simulink model "FAST_11TO14mpers_testIPC"  (R2019b)
settings: Solver=FixedStepAuto  StartTime=0.0  StopTime=400  FixedStep=DT  RelTol=1e-3
values from neighbouring files (symbols this model uses):
  Drivetrain = struct    [dataDLR.m]
  OutList = OutTable.Properties.VariableNames    [initLPVParam.m]    (also in testCtrl.m; testOutList.m = cell(40, 1); testqLPV.m = cell(40, 1))
undefined symbols (not defined in the file or in its folder): RPM_Init, strmatch
settings Model: ExtModeTrigMode=oneshot  ExtModeArmWhenConnect=off  Creator=Hazim Namik  LastModifiedBy=ditt_aj
settings DataIOCC: LimitDataPoints=on  SaveFormat=Array  ReturnWorkspaceOutputs=off
settings OptimizationCC: BlockReduction=off  BooleanDataType=off  LifeSpan=inf
settings DebuggingCC: SaveWithParameterizedLinksMsg=none  UnderspecifiedInitializationDetection=Classic  MergeDetectMultiDrivingBlocksExec=none  SignalResolutionControl=TryResolveAllWithWarning  SFUnexpectedBacktrackingDiag=warning  SFNoUnconditionalDefaultTransitionDiag=warning  SFExecutionAtInitializationDiag=none  ArithmeticOperatorsInVariantConditions=warning
settings HardwareCC: ProdBitPerPointer=32  ProdBitPerSizeT=32  ProdBitPerPtrDiffT=32  ProdLargestAtomicFloat=None  ProdIntDivRoundTo=Undefined  ProdEndianess=Unspecified  ProdWordSize=32  ProdHWDeviceType=32-bit Generic  TargetUnknown=on
settings ModelReferenceCC: PropagateSignalLabelsOutOfModel=off
settings SFSimCC: SimUseLocalCustomCode=off  CustomCodeUndefinedFunction=UseInterfaceOnly
settings RTWCC: RTWUseLocalCustomCode=off
settings CodeAppCC: StateflowObjectComments=on
settings GRTTargetCC: TargetLangStandard=C89/C90 (ANSI)  GeneratePreprocessorConditionals=Disable all
settings ConfigComp: CovMetricSettings=dw  CovHtmlReporting=on  CovSaveCumulativeToWorkspaceVar=on  CovSaveSingleToWorkspaceVar=on  CovExternalEMLEnable=off

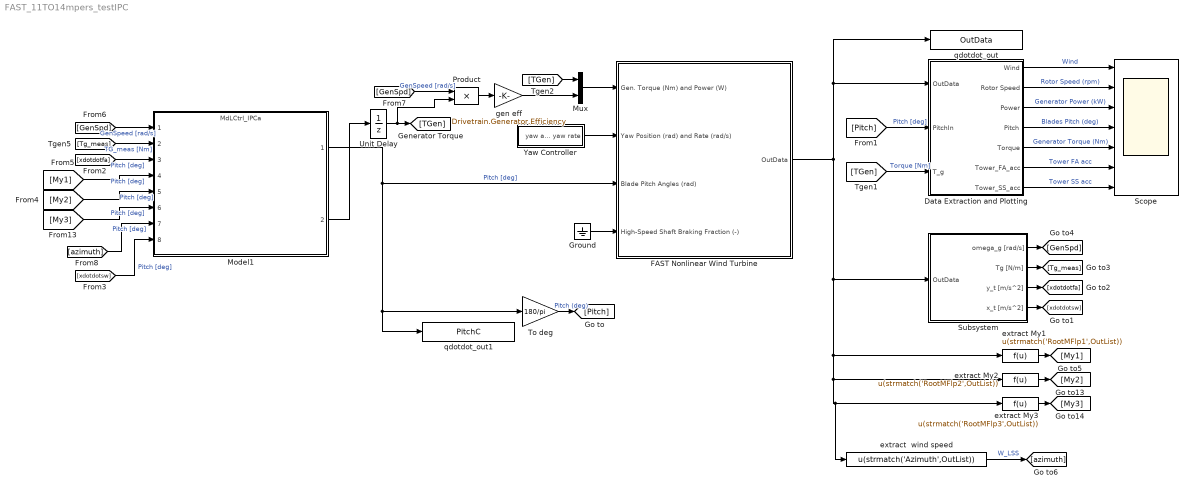
== system FAST_11TO14mpers_testIPC ==
  Data Extraction and Plotting : Subsystem
  FAST Nonlinear Wind Turbine : Subsystem  mask(FAST Nonlinear Wind Turbine){}
      mask help: This block contains the FAST S-Function.
      mask init:
      | clear FAST_SFunc
  Ground : Ground
  Model1 : ModelReference  ModelNameDialog=MdLCtrl_IPCa.slx  SimulationMode=Normal  ModelReferenceVersion=1.28
  Mux : Mux  Inputs=2
  Product : Product  RndMeth=Zero
  Scope : Scope  NumInputPorts=7
      settings: Tag=Scope
  Subsystem : Subsystem
  To deg : Gain  Gain=180/pi
  Unit Delay : UnitDelay  InitialCondition=RPM_Init*Drivetrain.Gearbox.Ratio  SampleTime=-1  HasFrameUpgradeWarning=on
  Yaw Controller : Subsystem
  extract  wind speed : Fcn  Expr=u(strmatch('Azimuth',OutList))
  extract My1 : Fcn  Expr=u(strmatch('RootMFlp1',OutList))
  extract My2 : Fcn  Expr=u(strmatch('RootMFlp2',OutList))
  extract My3 : Fcn  Expr=u(strmatch('RootMFlp3',OutList))
  gen eff : Gain  Gain=Drivetrain.Generator.Efficiency
  qdotdot_out : ToWorkspace  VariableName=OutData  SampleTime=-1
  qdotdot_out1 : ToWorkspace  VariableName=PitchC  SampleTime=-1
  wires:
  Mux/1 -> FAST Nonlinear Wind Turbine/1(Gen. Torque (Nm) and Power (W))
  Yaw Controller/1(yaw and yaw rate) -> FAST Nonlinear Wind Turbine/2(Yaw Position (rad) and Rate (rad/s))
  To deg/1 -> [Pitch]  "Pitch (deg)"
  gen eff/1 -> Mux/2
  Product/1 -> gen eff/1
  Data Extraction and Plotting/3(Power) -> Scope/3  "Generator Power (kW)"
  [Pitch] -> Data Extraction and Plotting/2(PitchIn)  "Pitch [deg]"
  Data Extraction and Plotting/1(Wind) -> Scope/1  "Wind"
  Data Extraction and Plotting/2(Rotor Speed) -> Scope/2  "Rotor Speed (rpm)"
  [TGen] -> Data Extraction and Plotting/3(T_g)  "Torque [Nm]"
  Data Extraction and Plotting/4(Pitch) -> Scope/4  "Blades Pitch (deg)"
  Data Extraction and Plotting/5(Torque) -> Scope/5  "Generator Torque (Nm)"
  Model1/2 -> Unit Delay/1
  Data Extraction and Plotting/6(Tower_FA_acc) -> Scope/6  "Tower FA acc"
  Data Extraction and Plotting/7(Tower_SS_acc) -> Scope/7  "Tower SS acc"
  Ground/1 -> FAST Nonlinear Wind Turbine/4(High-Speed Shaft Braking Fraction (-))
  [TGen] -> Mux/1
  Subsystem/1(omega_g [rad/s]) -> [GenSpd]
  Subsystem/3(y_t [m/s^2]) -> [xdotdotfa]
  Subsystem/4(x_t [m/s^2]) -> [xdotdotsw]
  [GenSpd] -> Model1/1  "GenSpeed [rad/s]"
  [Tg_meas] -> Model1/2  "TG_meas [Nm]"
  [xdotdotsw] -> Model1/8  "Pitch [deg]"
  [xdotdotfa] -> Model1/3  "Pitch [deg]"
  Subsystem/2(Tg [N/m]) -> [Tg_meas]
  [GenSpd] -> Product/1  "GenSpeed [rad/s]"
  Unit Delay/1 -> Product/2, [TGen]
  Model1/1 -> qdotdot_out1/1, To deg/1, FAST Nonlinear Wind Turbine/3(Blade Pitch Angles (rad))  "Pitch [deg]"
  FAST Nonlinear Wind Turbine/1(OutData) -> qdotdot_out/1, Data Extraction and Plotting/1(OutData), Subsystem/1(OutData), extract My1/1, extract My2/1, extract  wind speed/1, extract My3/1
  extract My2/1 -> [My2]
  extract My1/1 -> [My1]
  extract My3/1 -> [My3]
  [My1] -> Model1/4  "Pitch [deg]"
  [My2] -> Model1/5  "Pitch [deg]"
  [My3] -> Model1/6  "Pitch [deg]"
  extract  wind speed/1 -> [azimuth]  "W_LSS"
  [azimuth] -> Model1/7  "Pitch [deg]"

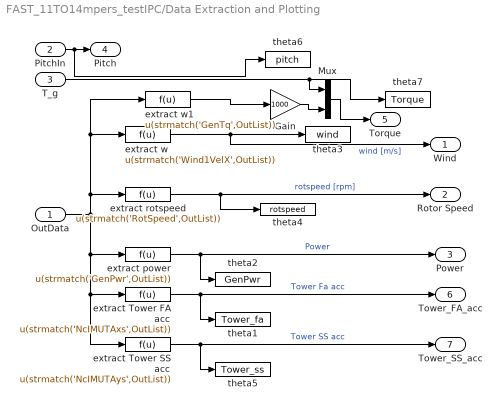
== system FAST_11TO14mpers_testIPC/Data Extraction and Plotting ==
  OutData : Inport
  PitchIn : Inport  Port=2
  T_g : Inport  Port=3
  Gain : Gain  Gain=1000
  Mux : Mux  Inputs=2
  extract Tower FA acc : Fcn  Expr=u(strmatch('NcIMUTAxs',OutList))
  extract Tower SS acc : Fcn  Expr=u(strmatch('NcIMUTAys',OutList))
  extract power : Fcn  Expr=u(strmatch('GenPwr',OutList))
  extract rotspeed : Fcn  Expr=u(strmatch('RotSpeed',OutList))
  extract w : Fcn  Expr=u(strmatch('Wind1VelX',OutList))
  extract w1 : Fcn  Expr=u(strmatch('GenTq',OutList))
  theta1 : ToWorkspace  VariableName=Tower_fa  SampleTime=-1
      settings: MaxDataPoints=Inf  Decimation=3
  theta2 : ToWorkspace  VariableName=GenPwr  SampleTime=-1
      settings: MaxDataPoints=Inf  Decimation=3
  theta3 : ToWorkspace  VariableName=wind  SampleTime=-1
      settings: MaxDataPoints=Inf  Decimation=3
  theta4 : ToWorkspace  VariableName=rotspeed  SampleTime=-1
      settings: MaxDataPoints=Inf  Decimation=3
  theta5 : ToWorkspace  VariableName=Tower_ss  SampleTime=-1
      settings: MaxDataPoints=Inf  Decimation=3
  theta6 : ToWorkspace  VariableName=pitch  SampleTime=-1
      settings: MaxDataPoints=Inf  Decimation=3
  theta7 : ToWorkspace  VariableName=Torque  SampleTime=-1
      settings: MaxDataPoints=Inf  Decimation=3
  Wind : Outport  VectorParamsAs1DForOutWhenUnconnected=off
  Rotor Speed : Outport  Port=2  VectorParamsAs1DForOutWhenUnconnected=off
  Power : Outport  Port=3  VectorParamsAs1DForOutWhenUnconnected=off
  Pitch : Outport  Port=4  VectorParamsAs1DForOutWhenUnconnected=off
  Torque : Outport  Port=5  VectorParamsAs1DForOutWhenUnconnected=off
  Tower_FA_acc : Outport  Port=6  VectorParamsAs1DForOutWhenUnconnected=off
  Tower_SS_acc : Outport  Port=7  VectorParamsAs1DForOutWhenUnconnected=off
  wires:
  extract w/1 -> Wind/1, theta3/1  "wind [m/s]"
  extract rotspeed/1 -> theta4/1, Rotor Speed/1  "rotspeed [rpm]"
  extract power/1 -> theta2/1, Power/1  "Power"
  PitchIn/1 -> theta6/1, Pitch/1
  T_g/1 -> Mux/1, theta7/1
  extract Tower FA acc/1 -> theta1/1, Tower_FA_acc/1  "Tower Fa acc"
  OutData/1 -> extract w/1, extract w1/1, extract rotspeed/1, extract Tower SS acc/1, extract Tower FA acc/1, extract power/1
  extract Tower SS acc/1 -> theta5/1, Tower_SS_acc/1  "Tower SS acc"
  extract w1/1 -> Gain/1
  Gain/1 -> Mux/2
  Mux/1 -> Torque/1

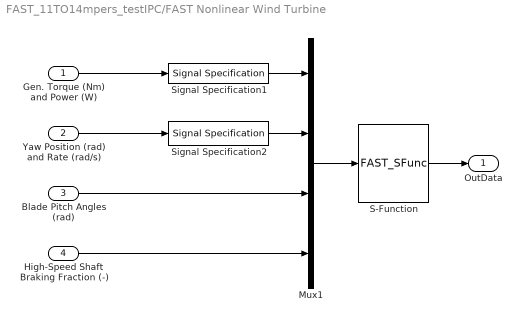
== system FAST_11TO14mpers_testIPC/FAST Nonlinear Wind Turbine ==
  Gen. Torque (Nm) and Power (W) : Inport
  Yaw Position (rad) and Rate (rad/s) : Inport  Port=2
  Blade Pitch Angles (rad) : Inport  Port=3
  High-Speed Shaft Braking Fraction (-) : Inport  Port=4
  Mux1 : Mux
  S-Function : S-Function  FunctionName=FAST_SFunc  Parameters=FAST_InputFileName, TMax, 0  SFunctionDeploymentMode=off  EnableBusSupport=off
  Signal Specification1 : SignalSpecification  OutDataTypeStr=double  Dimensions=2
  Signal Specification2 : SignalSpecification  OutDataTypeStr=double  Dimensions=2
  OutData : Outport  VectorParamsAs1DForOutWhenUnconnected=off
  wires:
  Gen. Torque (Nm) and Power (W)/1 -> Signal Specification1/1
  S-Function/1 -> OutData/1
  Mux1/1 -> S-Function/1
  Blade Pitch Angles (rad)/1 -> Mux1/3
  Yaw Position (rad) and Rate (rad/s)/1 -> Signal Specification2/1
  Signal Specification1/1 -> Mux1/1
  Signal Specification2/1 -> Mux1/2
  High-Speed Shaft Braking Fraction (-)/1 -> Mux1/4

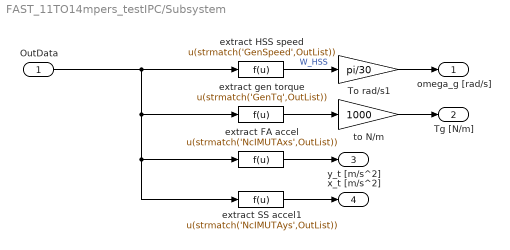
== system FAST_11TO14mpers_testIPC/Subsystem ==
  OutData : Inport
  To rad/s1 : Gain  Gain=pi/30
  extract FA accel : Fcn  Expr=u(strmatch('NcIMUTAxs',OutList))
  extract HSS speed : Fcn  Expr=u(strmatch('GenSpeed',OutList))
  extract SS accel1 : Fcn  Expr=u(strmatch('NcIMUTAys',OutList))
  extract gen torque : Fcn  Expr=u(strmatch('GenTq',OutList))
  to N/m : Gain  Gain=1000
  omega_g [rad/s] : Outport  VectorParamsAs1DForOutWhenUnconnected=off
  Tg [N/m] : Outport  Port=2  VectorParamsAs1DForOutWhenUnconnected=off
  y_t [m/s^2] : Outport  Port=3  VectorParamsAs1DForOutWhenUnconnected=off
  x_t [m/s^2] : Outport  Port=4  VectorParamsAs1DForOutWhenUnconnected=off
  wires:
  to N/m/1 -> Tg [N/m]/1
  OutData/1 -> extract SS accel1/1, extract FA accel/1, extract gen torque/1, extract HSS speed/1
  extract FA accel/1 -> y_t [m/s^2]/1
  extract HSS speed/1 -> To rad/s1/1  "W_HSS"
  extract gen torque/1 -> to N/m/1
  extract SS accel1/1 -> x_t [m/s^2]/1
  To rad/s1/1 -> omega_g [rad/s]/1

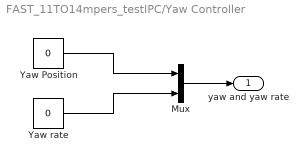
== system FAST_11TO14mpers_testIPC/Yaw Controller ==
  Mux : Mux  Inputs=2
  Yaw Position : Constant  Value=0
  Yaw rate : Constant  Value=0
  yaw and yaw rate : Outport  VectorParamsAs1DForOutWhenUnconnected=off
  wires:
  Mux/1 -> yaw and yaw rate/1
  Yaw Position/1 -> Mux/1
  Yaw rate/1 -> Mux/2
